simulink model "DSC"  (R2022b)
settings: Solver=FixedStepDiscrete  StartTime=0.0  StopTime=inf  FixedStep=0.05  RelTol=1e-3
PreLoadFcn:
  | canMessageBusType;
  | canFDMessageBusType;
values from neighbouring files (symbols this model uses):
  DSC_MODEL_CYCLE = 50.0    [DSC.sldd]
libraries: simulink x1, Mon3tr_Lib x1
PreSaveFcn:
  | filename = 'DSC';
  | dictionaryObj  = Simulink.data.dictionary.open([filename,'.sldd']);
  | saveChanges(dictionaryObj);
  | close(dictionaryObj);
  | disp([filename,'.sldd 已保存']);
settings Model: DataDictionary=DSC.sldd  Creator=Ligoo  LastModifiedBy=CENSORED
settings DataIOCC: SaveOutput=off  SignalLogging=off  DSMLogging=off  SaveTime=off  ReturnWorkspaceOutputs=off
settings OptimizationCC: DefaultParameterBehavior=Inlined  DefaultUnderspecifiedDataType=single  EnableMemcpy=off  ActiveStateOutputEnumStorageType=uint16  ZeroExternalMemoryAtStartup=off  ZeroInternalMemoryAtStartup=off  NoFixptDivByZeroProtection=on  EfficientFloat2IntCast=on  LifeSpan=Inf  MaxStackSize=200  OptimizeBlockOrder=speed  DifferentSizesBufferReuse=on  EfficientTunableParamExpr=on
settings DebuggingCC: SignalInfNanChecking=error  SignalRangeChecking=warning  AlgebraicLoopMsg=error  MergeDetectMultiDrivingBlocksExec=none  TasksWithSamePriorityMsg=error  IntegerOverflowMsg=error  UnconnectedInputMsg=error  UnconnectedOutputMsg=error  UnconnectedLineMsg=error  UniqueDataStoreMsg=warning  ModelReferenceIOMsg=error  ModelReferenceVersionMismatchMessage=error  StateNameClashWarn=warning  SFUnexpectedBacktrackingDiag=warning  SFNoUnconditionalDefaultTransitionDiag=warning  SFUndirectedBroadcastEventsDiag=error  IntegerSaturationMsg=error
settings HardwareCC: ProdBitPerPointer=32  ProdBitPerSizeT=32  ProdBitPerPtrDiffT=32  ProdLargestAtomicInteger=Long  ProdWordSize=32  ProdLongLongMode=on  ProdHWDeviceType=ARM Compatible->ARM 7
settings ModelReferenceCC: EnableRefExpFcnMdlSchedulingChecks=on
settings SFSimCC: MATLABDynamicMemAlloc=off
settings RTWCC: Description=Embedded Coder  SystemTargetFile=ert.tlc  GenCodeOnly=on  TemplateMakefile=ert_default_tmf  PostCodeGenCommand=FileCopy DSC  GenerateReport=on  RTWUseSimCustomCode=on  Toolchain=LCC-win64 v2.4.1 | gmake (64-bit Windows)  IncludeHyperlinkInReport=on  LaunchReport=on  GenerateTraceInfo=on  GenerateTraceReport=on  GenerateTraceReportSl=on  GenerateTraceReportSf=on  GenerateTraceReportEml=on
settings CodeAppCC: ForceParamTrailComments=on  IgnoreCustomStorageClasses=off  OperatorAnnotations=on  SimulinkDataObjDesc=on  SFDataObjDesc=on  MATLABFcnDesc=on  CustomSymbolStrUtil=$R$N$C  InsertBlockDesc=on  MATLABSourceComments=on
settings ERTTargetCC: MultiwordLength=2048  ConcurrentExecutionCompliant=off  IncludeMdlTerminateFcn=off  SuppressErrorStatus=on  SupportAbsoluteTime=off  SupportNonFinite=off  SupportComplex=off  ModelStepFunctionPrototypeControlCompliant=off  CPPClassGenCompliant=off  ArrayLayout=Row-major  GenerateASAP2=on  InlinedParameterPlacement=NonHierarchical  ERTCustomFileTemplate=example_file_process.tlc
settings ConfigComp: CovSaveCumulativeToWorkspaceVar=on  CovSaveSingleToWorkspaceVar=on  CovExternalEMLEnable=off  DVTestSuiteOptimization=CombinedObjectives (Nonlinear Extended)  DVDetectActiveLogic=on  DVModelReferenceHarness=on  DVHarnessSource=Signal Editor

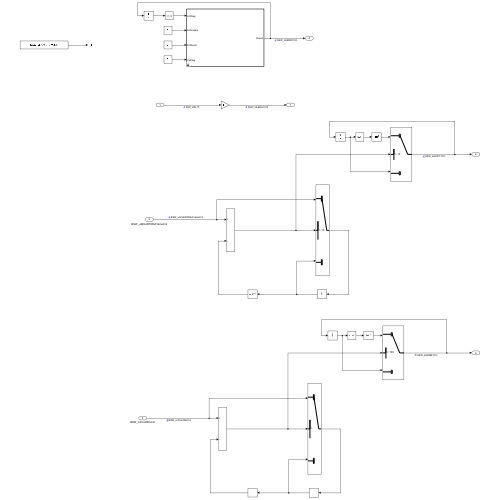
[thumbnail: Simulink's stored preview of the top-level diagram]
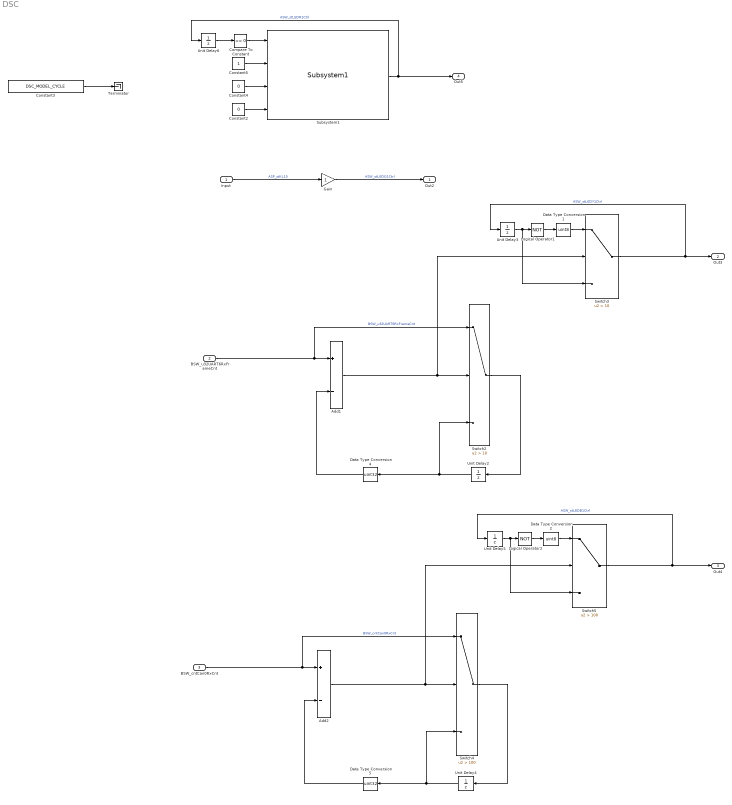
== system DSC ==
  Input : Inport
  BSW_u32UART6RxFrameCnt : Inport  Port=2
  BSW_cntCan0RxCnt : Inport  Port=3
  Add1 : Sum  Inputs=+-
  Add2 : Sum  Inputs=+-
  Compare To Constant : simulink/Logic and Bit Operations/Compare To Constant  relop===  const=0  OutDataTypeStr=uint8
  Constant2 : Constant  Value=0  OutDataTypeStr=uint8
  Constant3 : Constant  Value=DSC_MODEL_CYCLE
  Constant4 : Constant  Value=0  OutDataTypeStr=uint8
  Constant5 : Constant  OutDataTypeStr=uint8
  Data Type Conversion1 : DataTypeConversion  OutDataTypeStr=uint8  SaturateOnIntegerOverflow=off  RndMeth=Floor
  Data Type Conversion2 : DataTypeConversion  OutDataTypeStr=uint8  SaturateOnIntegerOverflow=off  RndMeth=Floor
  Data Type Conversion4 : DataTypeConversion  OutDataTypeStr=uint32  SaturateOnIntegerOverflow=off  RndMeth=Floor
  Data Type Conversion5 : DataTypeConversion  OutDataTypeStr=uint32  SaturateOnIntegerOverflow=off  RndMeth=Floor
  Gain : Gain  OutDataTypeStr=uint8
  Logical Operator1 : Logic  Operator=NOT  AllPortsSameDT=off  OutDataTypeStr=boolean
  Logical Operator2 : Logic  Operator=NOT  AllPortsSameDT=off  OutDataTypeStr=boolean
  Subsystem1 : Mon3tr_Lib/Subsystem1  Model_Cycle=DSC_MODEL_CYCLE  DiagEnable=uint8(1)  DiagDealTime=uint32(1000)  DiagHealTime=uint32(1000)  DiagDealTimeInit=uint32(0)  DiagHealType=uint8(0)
  Switch2 : Switch  Criteria=u2 > Threshold  Threshold=10  SaturateOnIntegerOverflow=off  InputSameDT=off
  Switch3 : Switch  Criteria=u2 > Threshold  Threshold=10  SaturateOnIntegerOverflow=off  InputSameDT=off
  Switch4 : Switch  Criteria=u2 > Threshold  Threshold=100  SaturateOnIntegerOverflow=off  InputSameDT=off
  Switch5 : Switch  Criteria=u2 > Threshold  Threshold=100  SaturateOnIntegerOverflow=off  InputSameDT=off
  Terminator : Terminator
  Unit Delay{2..6} (5 alike) : UnitDelay  SampleTime=-1  HasFrameUpgradeWarning=on
  Out2 : Outport
  Out3 : Outport  Port=2
  Out4 : Outport  Port=3
  Out5 : Outport  Port=4
  wires:
  Constant3/1 -> Terminator/1
  Input/1 -> Gain/1  "ASP_stKL15"
  Gain/1 -> Out2/1  "ASW_stLEDG1Ctrl"
  BSW_u32UART6RxFrameCnt/1 -> Switch2/1, Add1/1  "BSW_u32UART6RxFrameCnt"
  Unit Delay2/1 -> Switch2/3, Data Type Conversion4/1
  Switch2/1 -> Unit Delay2/1
  Switch3/1 -> Unit Delay3/1, Out3/1  "ASW_stLEDY1Ctrl"
  Logical Operator1/1 -> Data Type Conversion1/1
  Unit Delay3/1 -> Switch3/3, Logical Operator1/1
  Add1/1 -> Switch3/2, Switch2/2
  Data Type Conversion1/1 -> Switch3/1
  Add2/1 -> Switch5/2, Switch4/2
  Unit Delay4/1 -> Switch4/3, Data Type Conversion5/1
  Data Type Conversion2/1 -> Switch5/1
  Logical Operator2/1 -> Data Type Conversion2/1
  Unit Delay5/1 -> Switch5/3, Logical Operator2/1
  Switch5/1 -> Out4/1, Unit Delay5/1  "ASW_stLEDB1Ctrl"
  Switch4/1 -> Unit Delay4/1
  BSW_cntCan0RxCnt/1 -> Switch4/1, Add2/1  "BSW_cntCan0RxCnt"
  Data Type Conversion4/1 -> Add1/2
  Data Type Conversion5/1 -> Add2/2
  Constant2/1 -> Subsystem1/4
  Constant4/1 -> Subsystem1/3
  Constant5/1 -> Subsystem1/2
  Compare To Constant/1 -> Subsystem1/1
  Unit Delay6/1 -> Compare To Constant/1
  Subsystem1/1 -> Out5/1, Unit Delay6/1  "ASW_stLEDR1Ctrl"
